simulink model "ElectricVehicleThermalManagementWithHeatPump"  (R2024b)
settings: Solver=VariableStepAuto  StartTime=0.0  StopTime=3600  RelTol=1e-3  AbsTol=1e-3
PreLoadFcn:
  | init_nmpc
InitFcn:
  | init_nmpc
model workspace: external: MATLAB File ElectricVehicleThermalManagementWithHeatPumpParameters.m (data not in the file)
values from neighbouring files (symbols this model uses):
  battery_C1_LUT = [1913.6 12447 30609 ... (first row only)    [ElectricVehicleThermalManagementWithHeatPumpParameters.m]
  battery_capacity_LUT = [280.081 276.25 276.392]    [ElectricVehicleThermalManagementWithHeatPumpParameters.m]
  battery_cell_cp = 795    [ElectricVehicleThermalManagementWithHeatPumpParameters.m]
  battery_cell_mass = 2.5    [ElectricVehicleThermalManagementWithHeatPumpParameters.m]
  battery_Em_LUT = [3.4966 3.5057 3.5148 ... (first row only)    [ElectricVehicleThermalManagementWithHeatPumpParameters.m]
  battery_N_cells = 20    [ElectricVehicleThermalManagementWithHeatPumpParameters.m]
  battery_Qe_init = 0    [ElectricVehicleThermalManagementWithHeatPumpParameters.m]
  battery_R0_LUT = [0.0117 0.0085 0.009 ... (first row only)    [ElectricVehicleThermalManagementWithHeatPumpParameters.m]
  battery_R1_LUT = [0.0109 0.0029 0.0013 ... (first row only)    [ElectricVehicleThermalManagementWithHeatPumpParameters.m]
  battery_SOC_LUT = [0; 0.1; 0.25; 0.5; 0.75; 0.9; 1]    [ElectricVehicleThermalManagementWithHeatPumpParameters.m]
  battery_T_init = -10    [ElectricVehicleThermalManagementWithHeatPumpParameters.m]
  battery_temperature_LUT = [5 20 40]    [ElectricVehicleThermalManagementWithHeatPumpParameters.m]
  cabin_duct_area = 0.04    [ElectricVehicleThermalManagementWithHeatPumpParameters.m]
  cabin_T_init = -10    [ElectricVehicleThermalManagementWithHeatPumpParameters.m]
  chiller_area_primary = 0.43982297150257105    (= 0.439822971503)    [ElectricVehicleThermalManagementWithHeatPumpParameters.m]
  chiller_N_baffles = 3    [ElectricVehicleThermalManagementWithHeatPumpParameters.m]
  chiller_N_tubes = 100    [ElectricVehicleThermalManagementWithHeatPumpParameters.m]
  chiller_tube_D = 0.0035    [ElectricVehicleThermalManagementWithHeatPumpParameters.m]
  chiller_tube_L = 0.4    [ElectricVehicleThermalManagementWithHeatPumpParameters.m]
  chiller_wall_conductivity = 240    [ElectricVehicleThermalManagementWithHeatPumpParameters.m]
  chiller_wall_thickness = 0.0001    [ElectricVehicleThermalManagementWithHeatPumpParameters.m]
  cond_evap_air_area_flow = 0.3906    [ElectricVehicleThermalManagementWithHeatPumpParameters.m]
  cond_evap_air_area_primary = 1.4834999999999998    (= 1.4835)    [ElectricVehicleThermalManagementWithHeatPumpParameters.m]
  cond_evap_W = 0.015    [ElectricVehicleThermalManagementWithHeatPumpParameters.m]
  cond_evap_wall_conductivity = 240    [ElectricVehicleThermalManagementWithHeatPumpParameters.m]
  cond_evap_wall_thickness = 0.0001    [ElectricVehicleThermalManagementWithHeatPumpParameters.m]
  coolant_channel_D = 0.0092    [ElectricVehicleThermalManagementWithHeatPumpParameters.m]
  coolant_pipe_D = 0.019    [ElectricVehicleThermalManagementWithHeatPumpParameters.m]
  coolant_T_init = -10    [ElectricVehicleThermalManagementWithHeatPumpParameters.m]
  coolant_tank_area = 0.0121    [ElectricVehicleThermalManagementWithHeatPumpParameters.m]
  coolant_tank_volume = 1.25    [ElectricVehicleThermalManagementWithHeatPumpParameters.m]
  coolant_valve_D_ratio_max = 0.95    [ElectricVehicleThermalManagementWithHeatPumpParameters.m]
  coolant_valve_D_ratio_min = 0.001    [ElectricVehicleThermalManagementWithHeatPumpParameters.m]
  coolant_valve_displacement = 0.0063    [ElectricVehicleThermalManagementWithHeatPumpParameters.m]
  coolant_valve_S_max = 0.0053    [ElectricVehicleThermalManagementWithHeatPumpParameters.m]
  evaporator_air_area_flow = 0.12    [ElectricVehicleThermalManagementWithHeatPumpParameters.m]
  evaporator_air_area_primary = 0.4323    [ElectricVehicleThermalManagementWithHeatPumpParameters.m]
  evaporator_W = 0.015    [ElectricVehicleThermalManagementWithHeatPumpParameters.m]
  evaporator_wall_conductivity = 240    [ElectricVehicleThermalManagementWithHeatPumpParameters.m]
  evaporator_wall_thickness = 0.0001    [ElectricVehicleThermalManagementWithHeatPumpParameters.m]
  expansion_valve_D_ratio_max = 0.9    [ElectricVehicleThermalManagementWithHeatPumpParameters.m]
  hex_area_primary = 0.070371675440411369    (= 0.0703716754404)    [ElectricVehicleThermalManagementWithHeatPumpParameters.m]
  hex_N_tubes = 64    [ElectricVehicleThermalManagementWithHeatPumpParameters.m]
  hex_tube_D = 0.0035    [ElectricVehicleThermalManagementWithHeatPumpParameters.m]
  hex_wall_conductivity = 240    [ElectricVehicleThermalManagementWithHeatPumpParameters.m]
  hex_wall_thickness = 0.0001    [ElectricVehicleThermalManagementWithHeatPumpParameters.m]
  inner_cond_air_area_flow = 0.1953    [ElectricVehicleThermalManagementWithHeatPumpParameters.m]
  inner_cond_air_area_primary = 0.99520000000000008    (= 0.9952)    [ElectricVehicleThermalManagementWithHeatPumpParameters.m]
  inner_cond_W = 0.02    [ElectricVehicleThermalManagementWithHeatPumpParameters.m]
  inner_cond_wall_conductivity = 240    [ElectricVehicleThermalManagementWithHeatPumpParameters.m]
  inner_cond_wall_thickness = 0.0001    [ElectricVehicleThermalManagementWithHeatPumpParameters.m]
  pump_speed_max = 1000    [ElectricVehicleThermalManagementWithHeatPumpParameters.m]
  radiator_air_area_flow = 0.097499999999999989    (= 0.0975)    [ElectricVehicleThermalManagementWithHeatPumpParameters.m]
  radiator_air_area_primary = 0.43687499999999996    (= 0.436875)    [ElectricVehicleThermalManagementWithHeatPumpParameters.m]
  radiator_W = 0.015    [ElectricVehicleThermalManagementWithHeatPumpParameters.m]
  radiator_wall_conductivity = 240    [ElectricVehicleThermalManagementWithHeatPumpParameters.m]
  radiator_wall_thickness = 0.0001    [ElectricVehicleThermalManagementWithHeatPumpParameters.m]
  refrigerant_p_init = 0.2    [ElectricVehicleThermalManagementWithHeatPumpParameters.m]
  refrigerant_pipe_D = 0.01    [ElectricVehicleThermalManagementWithHeatPumpParameters.m]
  refrigerant_valve_D_ratio_max = 0.95    [ElectricVehicleThermalManagementWithHeatPumpParameters.m]
  refrigerant_valve_displacement = 0.005    [ElectricVehicleThermalManagementWithHeatPumpParameters.m]
libraries: fl_lib x227, nesl_utility x162, SimscapeFluids_lib x30, LiBatteryElements_lib x16, slpidlib x3, SignalEditorBlockLib x1
(part 9 of 13)

== system ElectricVehicleThermalManagementWithHeatPump/Controls/Compressor Control ==
  thermal_mode : Inport
  T_vent : Inport  Port=2
  T_vent_sp : Inport  Port=3
  p_low : Inport  Port=4
  p_high : Inport  Port=5
  Constant : Constant  Value=0
  Critical Cutoff : Lookup_n-D  NumberOfTableDimensions=1  BreakpointsForDimension1=[0 3.5 3.6 4]  IndexSearchMethod=Linear search  BeginIndexSearchUsingPreviousIndexResult=on  Table=[1 1 0 0]  ExtrapMethod=Clip  InternalRulePriority=Speed  RndMeth=Simplest
  Freezing Cutoff : Lookup_n-D  NumberOfTableDimensions=1  BreakpointsForDimension1=[0 0.05 0.15 0.3]  IndexSearchMethod=Linear search  BeginIndexSearchUsingPreviousIndexResult=on  Table=[0 0 1 1]  ExtrapMethod=Clip  InternalRulePriority=Speed  RndMeth=Simplest
  PI Controller Cooling : slpidlib/PID Controller  Controller=PI  Form=Parallel  TimeDomain=Continuous-time  UseExternalTs=off  SampleTime=-1  IntegratorMethod=Forward Euler  FilterMethod=Forward Euler  ControllerParametersSource=internal  P=0.05  I=0.005  UseKiTs=off  D=0  UseExternalDerivativeSource=off  N=100  UseFilter=on  TunerSelectOption=Transfer Function Based (PID Tuner App)  ZeroCross=off  InitialConditionSource=internal  InitialConditionForIntegrator=0  InitialConditionForFilter=0  DifferentiatorICPrevScaledInput=0  ExternalReset=either  TrackingMode=off  Kt=1  LimitOutput=on  SatLimitsSource=internal  UpperSaturationLimit=1  LowerSaturationLimit=0  LinearizeAsGain=on  AntiWindupMode=back-calculation  Kb=1  LimitIntegrator=off  UpperIntegratorSaturationLimit=inf  LowerIntegratorSaturationLimit=-inf  POutMin=[]  POutMax=[]  IOutMin=[]  IOutMax=[]  DOutMin=[]  DOutMax=[]  NOutMin=[]  NOutMax=[]  SumOutMin=[]  SumOutMax=[]  SaturationOutMin=[]  SaturationOutMax=[]  PParamMin=[]  PParamMax=[]  IParamMin=[]  IParamMax=[]  DParamMin=[]  DParamMax=[]  NParamMin=[]  NParamMax=[]  KbParamMin=[]  KbParamMax=[]  KtParamMin=[]  KtParamMax=[]  KbOutMin=[]  KbOutMax=[]  KtOutMin=[]  KtOutMax=[]  IntegratorOutMin=[]  IntegratorOutMax=[]  FilterOutMin=[]  FilterOutMax=[]  SumI1OutMin=[]  SumI1OutMax=[]  SumI2OutMin=[]  SumI2OutMax=[]  SumI3OutMin=[]  SumI3OutMax=[]  SumI4OutMin=[]  SumI4OutMax=[]  SumDOutMin=[]  SumDOutMax=[]  DifferentiatorOutMin=[]  DifferentiatorOutMax=[]  FilterDiffOutCoefMin=[]  FilterDiffOutCoefMax=[]  ReciprocalOutMin=[]  ReciprocalOutMax=[]  SumDenOutMin=[]  SumDenOutMax=[]  SumNumOutMin=[]  SumNumOutMax=[]  DivideOutMin=[]  DivideOutMax=[]  UdiffTsProdOutMin=[]  UdiffTsProdOutMax=[]  NTsProdOutMin=[]  NTsProdOutMax=[]  UintegralTsProdOutMin=[]  UintegralTsProdOutMax=[]  UngainTsProdOutMin=[]  UngainTsProdOutMax=[]  ClampingZeroOutDataTypeStr=Inherit: Inherit via back propagation  ClampingZeroOutMin=[]  ClampingZeroOutMax=[]  FilterDenConstantOutDataTypeStr=Inherit: Inherit via back propagation  FilterDenConstantOutMin=[]  FilterDenConstantOutMax=[]  PCopyOutDataTypeStr=Inherit: Inherit via back propagation  PCopyOutMin=[]  PCopyOutMax=[]  NCopyOutDataTypeStr=Inherit: Inherit via back propagation  NCopyOutMin=[]  NCopyOutMax=[]  IntegratorContinuousStateAttributes=''  IntegratorStateMustResolveToSignalObject=off  IntegratorRTWStateStorageClass=Auto  FilterContinuousStateAttributes=''  FilterStateMustResolveToSignalObject=off  FilterRTWStateStorageClass=Auto  ParallelPVariant=InternalParameters  IdealPVariant=Disabled  IVariant=InternalParameters  DVariant=Disabled  IntegratorVariant=Continuous  SatVariant=Enabled  AWVariant=BackCalculation  PCopyVariant=Disabled  TRVariant=Disabled  FdbkBlocksVariant=Forward  IdealPFdbkVariant=Disabled  SatFdbkVariant=Disabled  DerivativeFilterVariant=Disabled  NVariant=Disabled  NCopyVariant=Disabled_SignalSpec  FilterICVariant=Disabled  IntegratorICVariant=InternalICs  ExternalResetVariant=ExternalReset  TRSumVariant=Passthrough  SumFdbkVariant=Disabled  SumVariant=Sum_PI  TsampFilterVariant=InternalTs  TsampNgainVariant=Passthrough  TsampIntegralVariant=Disabled_SignalSpec  ExternalSaturationOutDataTypeStr=Inherit: Same as second input  DerivativeSourceVariant=Disabled  PreIntVariant=InternalPreInt
  PI Controller Heating : slpidlib/PID Controller  Controller=PI  Form=Parallel  TimeDomain=Continuous-time  UseExternalTs=off  SampleTime=-1  IntegratorMethod=Forward Euler  FilterMethod=Forward Euler  ControllerParametersSource=internal  P=-0.05  I=-0.005  UseKiTs=off  D=0  UseExternalDerivativeSource=off  N=100  UseFilter=on  TunerSelectOption=Transfer Function Based (PID Tuner App)  ZeroCross=off  InitialConditionSource=internal  InitialConditionForIntegrator=0  InitialConditionForFilter=0  DifferentiatorICPrevScaledInput=0  ExternalReset=either  TrackingMode=off  Kt=1  LimitOutput=on  SatLimitsSource=internal  UpperSaturationLimit=1  LowerSaturationLimit=0  LinearizeAsGain=on  AntiWindupMode=back-calculation  Kb=1  LimitIntegrator=off  UpperIntegratorSaturationLimit=inf  LowerIntegratorSaturationLimit=-inf  POutMin=[]  POutMax=[]  IOutMin=[]  IOutMax=[]  DOutMin=[]  DOutMax=[]  NOutMin=[]  NOutMax=[]  SumOutMin=[]  SumOutMax=[]  SaturationOutMin=[]  SaturationOutMax=[]  PParamMin=[]  PParamMax=[]  IParamMin=[]  IParamMax=[]  DParamMin=[]  DParamMax=[]  NParamMin=[]  NParamMax=[]  KbParamMin=[]  KbParamMax=[]  KtParamMin=[]  KtParamMax=[]  KbOutMin=[]  KbOutMax=[]  KtOutMin=[]  KtOutMax=[]  IntegratorOutMin=[]  IntegratorOutMax=[]  FilterOutMin=[]  FilterOutMax=[]  SumI1OutMin=[]  SumI1OutMax=[]  SumI2OutMin=[]  SumI2OutMax=[]  SumI3OutMin=[]  SumI3OutMax=[]  SumI4OutMin=[]  SumI4OutMax=[]  SumDOutMin=[]  SumDOutMax=[]  DifferentiatorOutMin=[]  DifferentiatorOutMax=[]  FilterDiffOutCoefMin=[]  FilterDiffOutCoefMax=[]  ReciprocalOutMin=[]  ReciprocalOutMax=[]  SumDenOutMin=[]  SumDenOutMax=[]  SumNumOutMin=[]  SumNumOutMax=[]  DivideOutMin=[]  DivideOutMax=[]  UdiffTsProdOutMin=[]  UdiffTsProdOutMax=[]  NTsProdOutMin=[]  NTsProdOutMax=[]  UintegralTsProdOutMin=[]  UintegralTsProdOutMax=[]  UngainTsProdOutMin=[]  UngainTsProdOutMax=[]  ClampingZeroOutDataTypeStr=Inherit: Inherit via back propagation  ClampingZeroOutMin=[]  ClampingZeroOutMax=[]  FilterDenConstantOutDataTypeStr=Inherit: Inherit via back propagation  FilterDenConstantOutMin=[]  FilterDenConstantOutMax=[]  PCopyOutDataTypeStr=Inherit: Inherit via back propagation  PCopyOutMin=[]  PCopyOutMax=[]  NCopyOutDataTypeStr=Inherit: Inherit via back propagation  NCopyOutMin=[]  NCopyOutMax=[]  IntegratorContinuousStateAttributes=''  IntegratorStateMustResolveToSignalObject=off  IntegratorRTWStateStorageClass=Auto  FilterContinuousStateAttributes=''  FilterStateMustResolveToSignalObject=off  FilterRTWStateStorageClass=Auto  ParallelPVariant=InternalParameters  IdealPVariant=Disabled  IVariant=InternalParameters  DVariant=Disabled  IntegratorVariant=Continuous  SatVariant=Enabled  AWVariant=BackCalculation  PCopyVariant=Disabled  TRVariant=Disabled  FdbkBlocksVariant=Forward  IdealPFdbkVariant=Disabled  SatFdbkVariant=Disabled  DerivativeFilterVariant=Disabled  NVariant=Disabled  NCopyVariant=Disabled_SignalSpec  FilterICVariant=Disabled  IntegratorICVariant=InternalICs  ExternalResetVariant=ExternalReset  TRSumVariant=Passthrough  SumFdbkVariant=Disabled  SumVariant=Sum_PI  TsampFilterVariant=InternalTs  TsampNgainVariant=Passthrough  TsampIntegralVariant=Disabled_SignalSpec  ExternalSaturationOutDataTypeStr=Inherit: Same as second input  DerivativeSourceVariant=Disabled  PreIntVariant=InternalPreInt
  Product : Product
  Product1 : Product
  Scope : Scope
  Scope1 : Scope
  Sum : Sum  Inputs=|+-
  Switch : Switch  Criteria=u2 > Threshold  Threshold=1  SaturateOnIntegerOverflow=off  InputSameDT=off
  Switch1 : Switch  Criteria=u2 > Threshold  SaturateOnIntegerOverflow=off  InputSameDT=off
  cmd_comp : Outport
  wires:
  p_low/1 -> Freezing Cutoff/1
  p_high/1 -> Critical Cutoff/1
  T_vent/1 -> Sum/1
  T_vent_sp/1 -> Sum/2
  Sum/1 -> PI Controller Cooling/1, PI Controller Heating/1
  PI Controller Heating/1 -> Switch/1
  PI Controller Cooling/1 -> Switch/3
  Switch1/1 -> cmd_comp/1
  Switch/1 -> Product1/1
  thermal_mode/1 -> Switch1/2, Switch/2, PI Controller Cooling/2, PI Controller Heating/2
  Freezing Cutoff/1 -> Scope1/1, Product/1
  Critical Cutoff/1 -> Scope/1, Product/2
  Product1/1 -> Switch1/1
  Constant/1 -> Switch1/3
  Product/1 -> Product1/2

== system ElectricVehicleThermalManagementWithHeatPump/Controls/Coolant Loop Control ==
  thermal_mode : Inport
  T_env : Inport  Port=2
  T_coolant_inverter_out : Inport  Port=3
  T_motor : Inport  Port=4
  T_battery : Inport  Port=5
  Battery Pump Control : Subsystem
  Motor Pump Control : Subsystem
  Parallel-Serial Mode : Subsystem
  To Workspace : ToWorkspace  VariableName=cmd_parallel_serial  SampleTime=-1
  cmd_parallel_serial : Outport
  cmd_motor_pump : Outport  Port=2
  cmd_battery_pump : Outport  Port=3
  wires:
  Parallel-Serial Mode/1(cmd_parallel_serial) -> To Workspace/1, cmd_parallel_serial/1, Battery Pump Control/3(cmd_parallel_serial)
  Motor Pump Control/1(cmd_motor_pump) -> cmd_motor_pump/1, Battery Pump Control/1(cmd_motor_pump)
  T_env/1 -> Parallel-Serial Mode/2(T_env)
  T_coolant_inverter_out/1 -> Parallel-Serial Mode/3(T_coolant_inverter_out)
  T_motor/1 -> Motor Pump Control/1(T_motor)
  Battery Pump Control/1(cmd_battery_pump) -> cmd_battery_pump/1
  T_battery/1 -> Battery Pump Control/2(T_battery)
  thermal_mode/1 -> Parallel-Serial Mode/1(thermal_mode)

== system ElectricVehicleThermalManagementWithHeatPump/Controls/Fan Control ==
  v_vehicle : Inport
  p_cond : Inport  Port=2
  T_env : Inport  Port=3
  cmd_comp : Inport  Port=4
  T_inverter : Inport  Port=5
  T_motor : Inport  Port=6
  2-D Lookup Table : Lookup_n-D  BreakpointsForDimension1=[0 1 2 3 4]  BreakpointsForDimension2=[0 1 2 3]  BeginIndexSearchUsingPreviousIndexResult=on  Table=[1 2 3 3; 0 1 3 3;0 0 2 3; 0 0 1 3; 0 0 0 3]  ExtrapMethod=Clip  InternalRulePriority=Speed  RndMeth=Simplest
      settings: InputPortMap=u0,u1
  Condenser Requirement : Subsystem
  Constant : Constant  Value=0
  Gain : Gain  Gain=1/3
  Inverter Requirement : Subsystem
  MinMax : MinMax  Function=max  Inputs=3
  Motor Requirement : Subsystem
  Scope{,1..3} (4 alike) : Scope
  Switch : Switch  Criteria=u2 > Threshold  SaturateOnIntegerOverflow=off  InputSameDT=off
  Vehicle Speed Requirement : Subsystem
  cmd_fan : Outport
  wires:
  T_motor/1 -> Motor Requirement/1(T_motor)
  T_inverter/1 -> Inverter Requirement/1(T_inverter)
  p_cond/1 -> Condenser Requirement/1(p_cond)
  T_env/1 -> Condenser Requirement/2(T_env)
  cmd_comp/1 -> Switch/2
  Constant/1 -> Switch/3
  Inverter Requirement/1(cmd_fan) -> Scope3/1, MinMax/2
  Switch/1 -> MinMax/1
  Motor Requirement/1(cmd_fan) -> Scope2/1, MinMax/3
  Vehicle Speed Requirement/1(req) -> 2-D Lookup Table/1
  Condenser Requirement/1(req) -> 2-D Lookup Table/2
  2-D Lookup Table/1 -> Gain/1
  Gain/1 -> Scope/1, Switch/1
  v_vehicle/1 -> Vehicle Speed Requirement/1(v_vehicle)
  MinMax/1 -> Scope1/1, cmd_fan/1

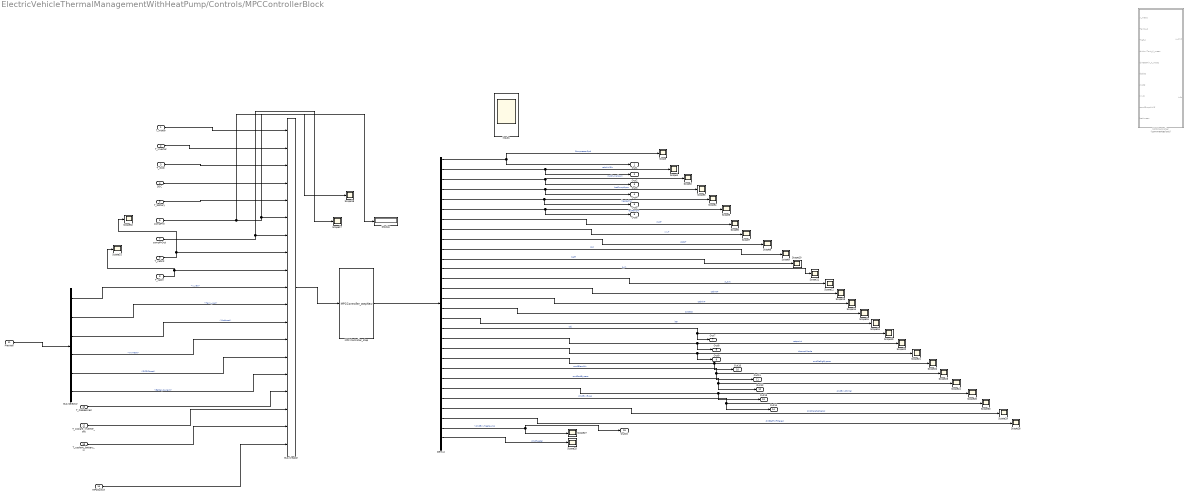
== system ElectricVehicleThermalManagementWithHeatPump/Controls/MPCControllerBlock ==
  T_motor : Inport
  T_inverter : Inport  Port=2
  T_dcdc : Inport  Port=3
  SOC : Inport  Port=4
  T_battery : Inport  Port=5
  compPrIn : Inport  Port=6
  compPrOut : Inport  Port=7
  T_cabInt : Inport  Port=8
  T_cabin : Inport  Port=9
  T_Cabdesired : Inport  Port=10
  Preview : Inport  Port=11
  T_coolant_inverter_out : Inport  Port=12
  T_coolant_battery_in : Inport  Port=13
  MPCSwitch : Inport  Port=14
  Bus Creator : BusCreator  Inputs=19
  Bus Selector : BusSelector  OutputSignals=v_vec,Tenv_vec,MotHeat,InvHeat,DCDCHeat,BatteryCurrent
  Demux : Demux  Outputs=30
  Display : Display
  "Inputs " : Scope
      settings: Floating=on
  MPC Controller_step : MATLABFcn  MATLABFcn=MPCController_stepNew  OutputDimensions=30
  MPCController : MATLAB Function  Commented=on  TreatAsAtomicUnit=on
  Scope{,1..32} (33 alike) : Scope
  Out1 : Outport
  Out2 : Outport  Port=2
  Out3 : Outport  Port=3
  Out4 : Outport  Port=4
  Out5 : Outport  Port=5
  Out6 : Outport  Port=6
  Out7 : Outport  Port=7
  Out8 : Outport  Port=8
  Out9 : Outport  Port=9
  Out10 : Outport  Port=10
  Out11 : Outport  Port=11
  Out12 : Outport  Port=12
  Out13 : Outport  Port=13
  Out14 : Outport  Port=14
  Out15 : Outport  Port=15
  wires:
  Bus Creator/1 -> MPC Controller_step/1
  T_Cabdesired/1 -> Bus Creator/16
  Preview/1 -> Bus Selector/1
  Bus Selector/2 -> Bus Creator/11  "<Tenv_vec>"
  Bus Selector/3 -> Bus Creator/12  "<MotHeat>"
  Bus Selector/4 -> Bus Creator/13  "<InvHeat>"
  Bus Selector/5 -> Bus Creator/14  "<DCDCHeat>"
  Bus Selector/6 -> Bus Creator/15  "<BatteryCurrent>"
  T_coolant_inverter_out/1 -> Bus Creator/17
  T_coolant_battery_in/1 -> Bus Creator/18
  T_motor/1 -> Bus Creator/1
  T_inverter/1 -> Bus Creator/2
  T_dcdc/1 -> Bus Creator/3
  SOC/1 -> Bus Creator/4
  T_battery/1 -> Bus Creator/5
  compPrIn/1 -> Scope18/1, Display/1, Bus Creator/6
  compPrOut/1 -> Scope17/1, Bus Creator/7
  T_cabInt/1 -> Scope32/1, Bus Creator/8
  T_cabin/1 -> Scope31/1, Bus Creator/9
  MPC Controller_step/1 -> Demux/1
  Demux/1 -> Out1/1, Scope/1  "CompressorSpd"
  Demux/2 -> Out2/1, Scope1/1  "cabAirMfIn"
  Demux/3 -> Out3/1, Scope2/1  "motPumpNrpm"
  Demux/4 -> Out4/1, Scope3/1  "batPumpNrpm"
  Demux/5 -> Out5/1, Scope4/1  "heaterPwr"
  Demux/6 -> Out6/1, Scope5/1  "radFanrpm"
  Demux/7 -> Scope6/1  "motT"
  Demux/8 -> Scope7/1  "invT"
  Demux/9 -> Scope8/1  "dcdcT"
  Demux/10 -> Scope9/1  "soc"
  Demux/11 -> Scope10/1  "batT"
  Demux/12 -> Scope11/1  "p_in"
  Demux/13 -> Scope12/1  "p_out"
  Demux/14 -> Scope13/1  "cabIntT"
  Demux/15 -> Scope14/1  "cabAirT"
  Demux/16 -> Scope15/1  "success"
  Demux/17 -> Scope16/1  "iter"
  Demux/18 -> Out7/1, Scope19/1  "obj"
  Demux/19 -> Out8/1, Scope20/1  "setpoint"
  Demux/20 -> Out9/1, Scope21/1  "thermalMode"
  Demux/21 -> Out10/1, Scope22/1  "cmdRefrigBypass"
  Demux/22 -> Out11/1, Scope23/1  "cmdBlendAir"
  Demux/23 -> Out12/1, Scope24/1  "cmdRadBypass"
  Demux/24 -> Out13/1, Scope26/1  "cmdExvChiller"
  Demux/29 -> Scope25/1  "cmdHeater"
  Demux/28 -> Scope27/1, Out15/1  "<cmdExvHeatpump"
  Demux/27 -> Scope28/1  "clntBatTinFiltered"
  Demux/26 -> Scope29/1  "cmdParallelSerial"
  Demux/25 -> Out14/1, Scope30/1  "cmdExvEvap"
  Bus Selector/1 -> Bus Creator/10  "<v_vec>"
  MPCSwitch/1 -> Bus Creator/19
